simulink library "lib_IC_GFM"  (R2026a)
settings: Solver=VariableStepAuto
undefined symbols (not defined in the file): block_buses, block_buses_DC, block_idx, block_toM, buses_lf, fb, fref, iC, invL, iR, iTf, Kic, Kiv, Kpc, Kpv, Nbuses_DC, omegab, op_intconv_GFM
libraries: simulink x4, sl_discontinuities x2
(part 2 of 2)

== system lib_IC_GFM/intconv_GFM/VCC/dynamic/RC/static omega ==
  i_d_in : Inport
  i_d_out : Inport  Port=2
  i_q_in : Inport  Port=3
  i_q_out : Inport  Port=4
  Gain : Gain  Gain=1./(iR.^2+C.^2)
  Gain2 : Gain  Gain=1./(iR.^2+C.^2)
  Gain3 : Gain  Gain=iR
  Gain4 : Gain  Gain=C
  Gain5 : Gain  Gain=iR
  Gain6 : Gain  Gain=C
  Sum : Sum  Inputs=|++
  Sum1 : Sum  Inputs=|+-
  Sum2 : Sum  Inputs=|+-
  Sum4 : Sum  Inputs=|-+
  v_d : Outport
  v_q : Outport  Port=2
  wires:
  Sum/1 -> v_d/1
  Sum4/1 -> v_q/1
  Gain5/1 -> Sum4/2
  Gain4/1 -> Sum4/1
  Gain6/1 -> Sum/2
  Gain3/1 -> Sum/1
  Gain2/1 -> Gain5/1, Gain6/1
  Gain/1 -> Gain3/1, Gain4/1
  i_d_out/1 -> Sum1/2
  i_d_in/1 -> Sum1/1  "id"
  i_q_out/1 -> Sum2/2  "iq2"
  Sum2/1 -> Gain2/1  "iq"
  Sum1/1 -> Gain/1  "id"
  i_q_in/1 -> Sum2/1  "iq1"

== system lib_IC_GFM/intconv_GFM/VCC/dynamic/RL/dynamic ==
  v_in_d : Inport
  v_out_d : Inport  Port=2
  v_in_q : Inport  Port=3
  v_out_q : Inport  Port=4
  Gain1 : Gain  Gain=L
  Gain2 : Gain  Gain=R
  Gain3 : Gain  Gain=R
  Gain4 : Gain  Gain=L
  Gain5 : Gain  Gain=invL.*omegab
  Gain7 : Gain  Gain=invL.*omegab
  Product : Product
  Product1 : Product
  Sum4 : Sum  Inputs=+-|
  Sum5 : Sum  Inputs=|-+
  Sum6 : Sum  Inputs=|++
  Sum7 : Sum  Inputs=-+|
  Sum8 : Sum  Inputs=|+-
  Sum9 : Sum  Inputs=-+|
  i_d : Integrator  InitialCondition=op_intconv_GFM.VCC_dynamic_RL_dynamic_i_d
  i_q : Integrator  InitialCondition=op_intconv_GFM.VCC_dynamic_RL_dynamic_i_q
  id : Outport
  iq : Outport  Port=2
  wires:
  v_in_q/1 -> Sum5/2  "v_in_q"
  v_in_d/1 -> Sum4/1  "v_in_d"
  Gain2/1 -> Sum4/2
  i_d/1 -> Gain2/1, Gain1/1, id/1  "id"
  Sum6/1 -> Gain5/1
  [omega_ref] -> Product1/1, Product/2  "omega"
  Gain5/1 -> i_d/1
  Product/1 -> Sum6/2
  Sum8/1 -> Gain7/1
  Sum4/1 -> Sum7/2
  Product1/1 -> Sum8/2
  Gain4/1 -> Product/1
  Sum7/1 -> Sum6/1
  Gain3/1 -> Sum5/1
  Sum5/1 -> Sum9/2
  Gain7/1 -> i_q/1
  i_q/1 -> Gain3/1, Gain4/1, iq/1  "iq"
  Gain1/1 -> Product1/2
  Sum9/1 -> Sum8/1
  v_out_d/1 -> Sum7/1  "v_out_d"
  v_out_q/1 -> Sum9/1  "v_out_q"

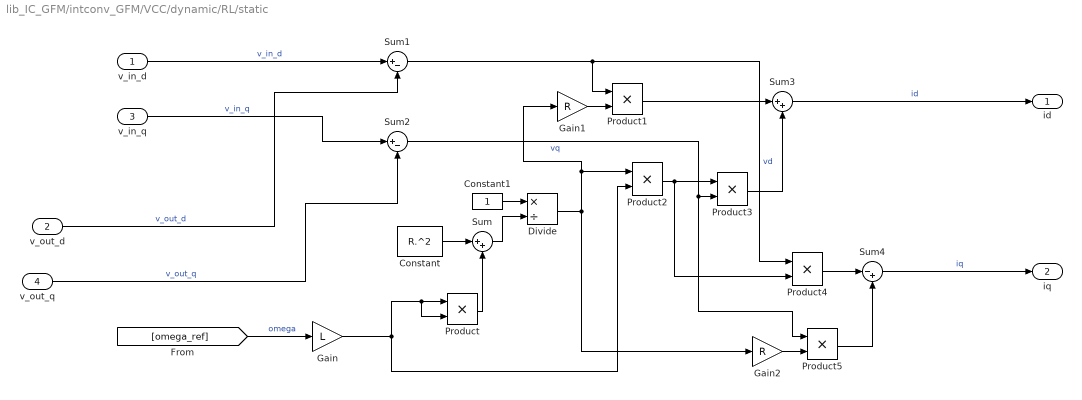
== system lib_IC_GFM/intconv_GFM/VCC/dynamic/RL/static ==
  v_in_d : Inport
  v_out_d : Inport  Port=2
  v_in_q : Inport  Port=3
  v_out_q : Inport  Port=4
  Constant : Constant  Value=R.^2
  Constant1 : Constant
  Divide : Product  Inputs=*/
  Gain : Gain  Gain=L
  Gain1 : Gain  Gain=R
  Gain2 : Gain  Gain=R
  Product{,1..5} (6 alike) : Product
  Sum : Sum  Inputs=|++
  Sum1 : Sum  Inputs=|+-
  Sum2 : Sum  Inputs=|+-
  Sum3 : Sum  Inputs=|++
  Sum4 : Sum  Inputs=|-+
  id : Outport
  iq : Outport  Port=2
  wires:
  v_in_q/1 -> Sum2/1  "v_in_q"
  v_out_d/1 -> Sum1/2  "v_out_d"
  Sum/1 -> Divide/2
  Gain2/1 -> Product5/2
  Product/1 -> Sum/2
  Product1/1 -> Sum3/1
  Product5/1 -> Sum4/2
  Constant/1 -> Sum/1
  Sum2/1 -> Product3/2, Product5/1  "vq"
  Gain/1 -> Product2/2, Product/1, Product/2
  Constant1/1 -> Divide/1
  Product3/1 -> Sum3/2
  Sum1/1 -> Product4/1, Product1/1  "vd"
  Divide/1 -> Product2/1, Gain1/1, Gain2/1
  Product4/1 -> Sum4/1
  Product2/1 -> Product3/1, Product4/2
  Gain1/1 -> Product1/2
  Sum3/1 -> id/1  "id"
  Sum4/1 -> iq/1  "iq"
  v_out_q/1 -> Sum2/2  "v_out_q"
  v_in_d/1 -> Sum1/1  "v_in_d"
  [omega_ref] -> Gain/1  "omega"

== system lib_IC_GFM/intconv_GFM/VCC/dynamic/RL/static_omega ==
  v_in_d : Inport
  v_out_d : Inport  Port=2
  v_in_q : Inport  Port=3
  v_out_q : Inport  Port=4
  Gain : Gain  Gain=1./(R.^2+L.^2)
  Gain2 : Gain  Gain=1./(R.^2+L.^2)
  Gain3 : Gain  Gain=R
  Gain4 : Gain  Gain=L
  Gain5 : Gain  Gain=L
  Gain6 : Gain  Gain=R
  Sum : Sum  Inputs=|++
  Sum1 : Sum  Inputs=|+-
  Sum2 : Sum  Inputs=|+-
  Sum3 : Sum  Inputs=|-+
  id : Outport
  iq : Outport  Port=2
  wires:
  Gain6/1 -> Sum3/2
  Sum3/1 -> iq/1
  Gain5/1 -> Sum3/1
  Sum/1 -> id/1
  Gain2/1 -> Gain4/1, Gain6/1
  Gain4/1 -> Sum/2
  Gain3/1 -> Sum/1
  Gain/1 -> Gain3/1, Gain5/1
  Sum2/1 -> Gain2/1  "vq"
  Sum1/1 -> Gain/1  "vd"
  v_out_d/1 -> Sum1/2  "v_out_d"
  v_out_q/1 -> Sum2/2  "v_out_q"
  v_in_d/1 -> Sum1/1  "v_in_d"
  v_in_q/1 -> Sum2/1  "v_in_q"

== system lib_IC_GFM/intconv_GFM/VCC/dynamic_VC/RC/dynamic ==
  omega : Inport
  i_d_in : Inport  Port=2
  i_d_out : Inport  Port=3
  i_q_in : Inport  Port=4
  i_q_out : Inport  Port=5
  Gain1 : Gain  Gain=iR
  Gain2 : Gain  Gain=iR
  Gain3 : Gain  Gain=C
  Gain4 : Gain  Gain=C
  Gain5 : Gain  Gain=iC.*omegab
  Gain6 : Gain  Gain=iC.*omegab
  Product : Product
  Product1 : Product
  Sum10 : Sum  Inputs=|-++
  Sum11 : Sum  Inputs=-+|
  Sum12 : Sum  Inputs=|+-
  Sum13 : Sum  Inputs=-+-|
  vd : Integrator  InitialCondition=op_intconv_GFM.VCC_dynamic_VC_RC_dynamic_vd
  vq : Integrator  InitialCondition=op_intconv_GFM.VCC_dynamic_VC_RC_dynamic_vq
  v_d : Outport
  v_q : Outport  Port=2
  wires:
  i_q_out/1 -> Sum12/2  "iq2"
  i_q_in/1 -> Sum12/1  "iq1"
  i_d_out/1 -> Sum11/1  "id2"
  i_d_in/1 -> Sum11/2  "id1"
  vd/1 -> Gain1/1, v_d/1, Gain4/1  "vd"
  Sum12/1 -> Sum13/2
  Gain5/1 -> vq/1
  Gain1/1 -> Sum10/1
  Sum13/1 -> Gain5/1
  omega/1 -> Product1/2, Product/2  "omega"
  Gain6/1 -> vd/1
  Sum11/1 -> Sum10/2
  Product/1 -> Sum13/1
  Gain2/1 -> Sum13/3
  Gain4/1 -> Product/1
  Product1/1 -> Sum10/3
  vq/1 -> Gain3/1, Gain2/1, v_q/1  "vq"
  Gain3/1 -> Product1/1
  Sum10/1 -> Gain6/1

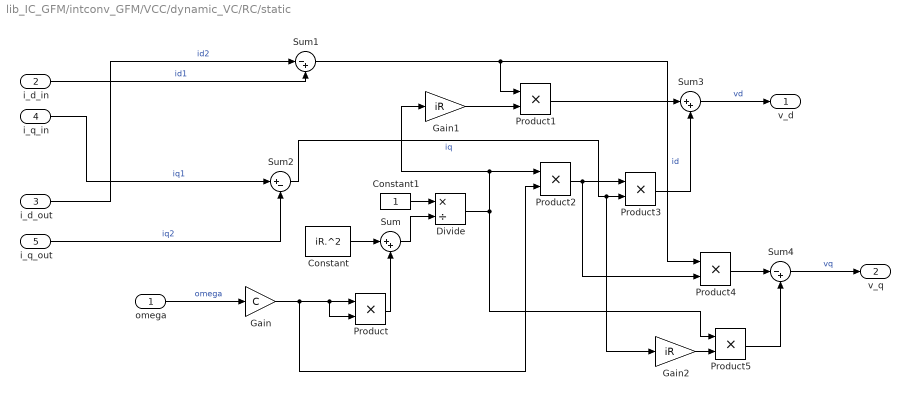
== system lib_IC_GFM/intconv_GFM/VCC/dynamic_VC/RC/static ==
  omega : Inport
  i_d_in : Inport  Port=2
  i_d_out : Inport  Port=3
  i_q_in : Inport  Port=4
  i_q_out : Inport  Port=5
  Constant : Constant  Value=iR.^2
  Constant1 : Constant
  Divide : Product  Inputs=*/
  Gain : Gain  Gain=C
  Gain1 : Gain  Gain=iR
  Gain2 : Gain  Gain=iR
  Product{,1..5} (6 alike) : Product
  Sum : Sum  Inputs=|++
  Sum1 : Sum  Inputs=|-+
  Sum2 : Sum  Inputs=|+-
  Sum3 : Sum  Inputs=|++
  Sum4 : Sum  Inputs=|-+
  v_d : Outport
  v_q : Outport  Port=2
  wires:
  i_q_out/1 -> Sum2/2  "iq2"
  i_q_in/1 -> Sum2/1  "iq1"
  i_d_out/1 -> Sum1/1  "id2"
  i_d_in/1 -> Sum1/2  "id1"
  omega/1 -> Gain/1  "omega"
  Sum3/1 -> v_d/1  "vd"
  Sum4/1 -> v_q/1  "vq"
  Constant/1 -> Sum/1
  Sum/1 -> Divide/2
  Gain/1 -> Product2/2, Product/2, Product/1
  Product/1 -> Sum/2
  Constant1/1 -> Divide/1
  Sum1/1 -> Product1/1, Product4/1  "id"
  Sum2/1 -> Gain2/1, Product3/2  "iq"
  Gain1/1 -> Product1/2
  Divide/1 -> Product5/1, Gain1/1, Product2/1
  Product1/1 -> Sum3/1
  Product3/1 -> Sum3/2
  Product2/1 -> Product4/2, Product3/1
  Product4/1 -> Sum4/1
  Gain2/1 -> Product5/2
  Product5/1 -> Sum4/2

== system lib_IC_GFM/intconv_GFM/VCC/dynamic_VC/RC/static omega ==
  i_d_in : Inport
  i_d_out : Inport  Port=2
  i_q_in : Inport  Port=3
  i_q_out : Inport  Port=4
  Gain : Gain  Gain=1./(iR.^2+C.^2)
  Gain2 : Gain  Gain=1./(iR.^2+C.^2)
  Gain3 : Gain  Gain=iR
  Gain4 : Gain  Gain=C
  Gain5 : Gain  Gain=iR
  Gain6 : Gain  Gain=C
  Sum : Sum  Inputs=|++
  Sum1 : Sum  Inputs=|+-
  Sum2 : Sum  Inputs=|+-
  Sum4 : Sum  Inputs=|-+
  v_d : Outport
  v_q : Outport  Port=2
  wires:
  Sum/1 -> v_d/1
  Sum4/1 -> v_q/1
  Gain5/1 -> Sum4/2
  Gain4/1 -> Sum4/1
  Gain6/1 -> Sum/2
  Gain3/1 -> Sum/1
  Gain2/1 -> Gain5/1, Gain6/1
  Gain/1 -> Gain3/1, Gain4/1
  i_d_out/1 -> Sum1/2
  i_d_in/1 -> Sum1/1  "id"
  i_q_out/1 -> Sum2/2  "iq2"
  Sum2/1 -> Gain2/1  "iq"
  Sum1/1 -> Gain/1  "id"
  i_q_in/1 -> Sum2/1  "iq1"

== system lib_IC_GFM/intconv_GFM/VCC/dynamic_limiting/RC/dynamic ==
  omega : Inport
  i_d_in : Inport  Port=2
  i_d_out : Inport  Port=3
  i_q_in : Inport  Port=4
  i_q_out : Inport  Port=5
  Gain1 : Gain  Gain=iR
  Gain2 : Gain  Gain=iR
  Gain3 : Gain  Gain=C
  Gain4 : Gain  Gain=C
  Gain5 : Gain  Gain=iC.*omegab
  Gain6 : Gain  Gain=iC.*omegab
  Product : Product
  Product1 : Product
  Sum10 : Sum  Inputs=|-++
  Sum11 : Sum  Inputs=-+|
  Sum12 : Sum  Inputs=|+-
  Sum13 : Sum  Inputs=-+-|
  vd : Integrator  InitialCondition=op_intconv_GFM.VCC_dynamic_limiting_RC_dynamic_vd
  vq : Integrator  InitialCondition=op_intconv_GFM.VCC_dynamic_limiting_RC_dynamic_vq
  v_d : Outport
  v_q : Outport  Port=2
  wires:
  Sum10/1 -> Gain6/1
  Gain3/1 -> Product1/1
  vq/1 -> v_q/1, Gain2/1, Gain3/1  "vq"
  Product1/1 -> Sum10/3
  Gain4/1 -> Product/1
  Gain2/1 -> Sum13/3
  Product/1 -> Sum13/1
  Sum11/1 -> Sum10/2
  Gain6/1 -> vd/1
  omega/1 -> Product/2, Product1/2  "omega"
  Sum13/1 -> Gain5/1
  Gain1/1 -> Sum10/1
  Gain5/1 -> vq/1
  Sum12/1 -> Sum13/2
  vd/1 -> Gain4/1, v_d/1, Gain1/1  "vd"
  i_d_in/1 -> Sum11/2  "id1"
  i_d_out/1 -> Sum11/1  "id2"
  i_q_in/1 -> Sum12/1  "iq1"
  i_q_out/1 -> Sum12/2  "iq2"

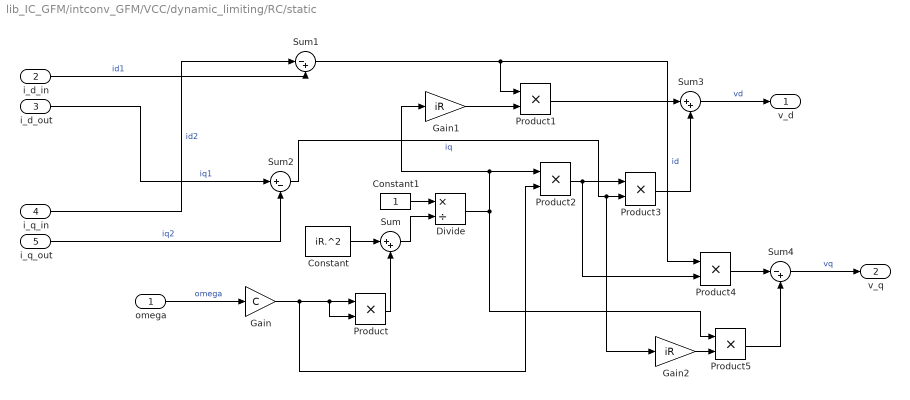
== system lib_IC_GFM/intconv_GFM/VCC/dynamic_limiting/RC/static ==
  omega : Inport
  i_d_in : Inport  Port=2
  i_d_out : Inport  Port=3
  i_q_in : Inport  Port=4
  i_q_out : Inport  Port=5
  Constant : Constant  Value=iR.^2
  Constant1 : Constant
  Divide : Product  Inputs=*/
  Gain : Gain  Gain=C
  Gain1 : Gain  Gain=iR
  Gain2 : Gain  Gain=iR
  Product{,1..5} (6 alike) : Product
  Sum : Sum  Inputs=|++
  Sum1 : Sum  Inputs=|-+
  Sum2 : Sum  Inputs=|+-
  Sum3 : Sum  Inputs=|++
  Sum4 : Sum  Inputs=|-+
  v_d : Outport
  v_q : Outport  Port=2
  wires:
  Product5/1 -> Sum4/2
  Gain2/1 -> Product5/2
  Product4/1 -> Sum4/1
  Product2/1 -> Product3/1, Product4/2
  Product3/1 -> Sum3/2
  Product1/1 -> Sum3/1
  Divide/1 -> Product2/1, Gain1/1, Product5/1
  Gain1/1 -> Product1/2
  Sum2/1 -> Product3/2, Gain2/1  "iq"
  Sum1/1 -> Product4/1, Product1/1  "id"
  Constant1/1 -> Divide/1
  Product/1 -> Sum/2
  Gain/1 -> Product/1, Product/2, Product2/2
  Sum/1 -> Divide/2
  Constant/1 -> Sum/1
  Sum4/1 -> v_q/1  "vq"
  Sum3/1 -> v_d/1  "vd"
  omega/1 -> Gain/1  "omega"
  i_d_in/1 -> Sum1/2  "id1"
  i_q_in/1 -> Sum1/1  "id2"
  i_d_out/1 -> Sum2/1  "iq1"
  i_q_out/1 -> Sum2/2  "iq2"

== system lib_IC_GFM/intconv_GFM/VCC/dynamic_limiting/RC/static omega ==
  i_d_in : Inport
  i_d_out : Inport  Port=2
  i_q_in : Inport  Port=3
  i_q_out : Inport  Port=4
  Gain : Gain  Gain=1./(iR.^2+C.^2)
  Gain2 : Gain  Gain=1./(iR.^2+C.^2)
  Gain3 : Gain  Gain=iR
  Gain4 : Gain  Gain=C
  Gain5 : Gain  Gain=iR
  Gain6 : Gain  Gain=C
  Sum : Sum  Inputs=|++
  Sum1 : Sum  Inputs=|+-
  Sum2 : Sum  Inputs=|+-
  Sum4 : Sum  Inputs=|-+
  v_d : Outport
  v_q : Outport  Port=2
  wires:
  i_q_in/1 -> Sum2/1  "iq1"
  Sum1/1 -> Gain/1  "id"
  Sum2/1 -> Gain2/1  "iq"
  i_q_out/1 -> Sum2/2  "iq2"
  i_d_in/1 -> Sum1/1  "id"
  i_d_out/1 -> Sum1/2
  Gain/1 -> Gain4/1, Gain3/1
  Gain2/1 -> Gain6/1, Gain5/1
  Gain3/1 -> Sum/1
  Gain6/1 -> Sum/2
  Gain4/1 -> Sum4/1
  Gain5/1 -> Sum4/2
  Sum4/1 -> v_q/1
  Sum/1 -> v_d/1

== system lib_IC_GFM/intconv_GFM/VCC/dynamic_limiting/RL/dynamic ==
  v_in_d : Inport
  v_out_d : Inport  Port=2
  v_in_q : Inport  Port=3
  v_out_q : Inport  Port=4
  Gain1 : Gain  Gain=L
  Gain2 : Gain  Gain=R
  Gain3 : Gain  Gain=R
  Gain4 : Gain  Gain=L
  Gain5 : Gain  Gain=invL.*omegab
  Gain7 : Gain  Gain=invL.*omegab
  Product : Product
  Product1 : Product
  Sum4 : Sum  Inputs=+-|
  Sum5 : Sum  Inputs=|-+
  Sum6 : Sum  Inputs=|++
  Sum7 : Sum  Inputs=-+|
  Sum8 : Sum  Inputs=|+-
  Sum9 : Sum  Inputs=-+|
  i_d : Integrator  InitialCondition=op_intconv_GFM.VCC_dynamic_limiting_RL_dynamic_i_d
  i_q : Integrator  InitialCondition=op_intconv_GFM.VCC_dynamic_limiting_RL_dynamic_i_q
  id : Outport
  iq : Outport  Port=2
  wires:
  v_out_q/1 -> Sum9/1  "v_out_q"
  v_out_d/1 -> Sum7/1  "v_out_d"
  Sum9/1 -> Sum8/1
  Gain1/1 -> Product1/2
  i_q/1 -> iq/1, Gain4/1, Gain3/1  "iq"
  Gain7/1 -> i_q/1
  Sum5/1 -> Sum9/2
  Gain3/1 -> Sum5/1
  Sum7/1 -> Sum6/1
  Gain4/1 -> Product/1
  Product1/1 -> Sum8/2
  Sum4/1 -> Sum7/2
  Sum8/1 -> Gain7/1
  Product/1 -> Sum6/2
  Gain5/1 -> i_d/1
  [omega_leader_VCVSC] -> Product/2, Product1/1  "omega"
  Sum6/1 -> Gain5/1
  i_d/1 -> id/1, Gain1/1, Gain2/1  "id"
  Gain2/1 -> Sum4/2
  v_in_d/1 -> Sum4/1  "v_in_d"
  v_in_q/1 -> Sum5/2  "v_in_q"

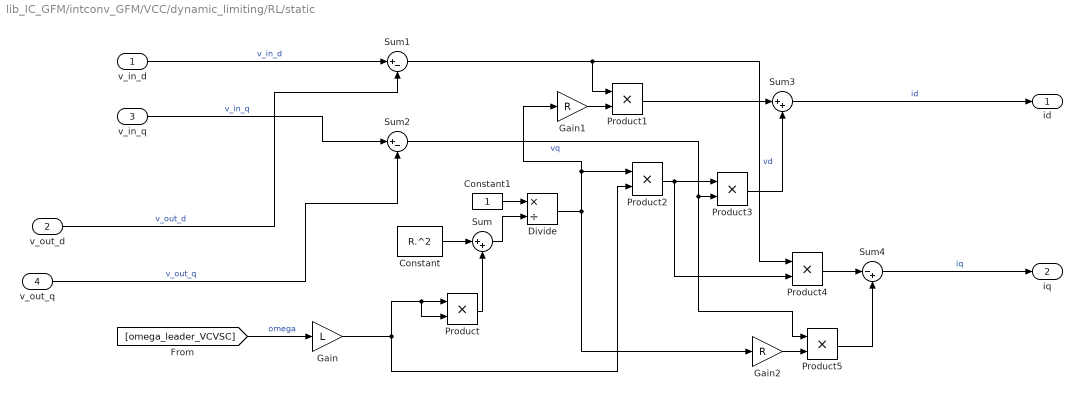
== system lib_IC_GFM/intconv_GFM/VCC/dynamic_limiting/RL/static ==
  v_in_d : Inport
  v_out_d : Inport  Port=2
  v_in_q : Inport  Port=3
  v_out_q : Inport  Port=4
  Constant : Constant  Value=R.^2
  Constant1 : Constant
  Divide : Product  Inputs=*/
  Gain : Gain  Gain=L
  Gain1 : Gain  Gain=R
  Gain2 : Gain  Gain=R
  Product{,1..5} (6 alike) : Product
  Sum : Sum  Inputs=|++
  Sum1 : Sum  Inputs=|+-
  Sum2 : Sum  Inputs=|+-
  Sum3 : Sum  Inputs=|++
  Sum4 : Sum  Inputs=|-+
  id : Outport
  iq : Outport  Port=2
  wires:
  [omega_leader_VCVSC] -> Gain/1  "omega"
  v_in_d/1 -> Sum1/1  "v_in_d"
  v_out_q/1 -> Sum2/2  "v_out_q"
  Sum4/1 -> iq/1  "iq"
  Sum3/1 -> id/1  "id"
  Gain1/1 -> Product1/2
  Product2/1 -> Product4/2, Product3/1
  Product4/1 -> Sum4/1
  Divide/1 -> Gain2/1, Gain1/1, Product2/1
  Sum1/1 -> Product1/1, Product4/1  "vd"
  Product3/1 -> Sum3/2
  Constant1/1 -> Divide/1
  Gain/1 -> Product/2, Product/1, Product2/2
  Sum2/1 -> Product5/1, Product3/2  "vq"
  Constant/1 -> Sum/1
  Product5/1 -> Sum4/2
  Product1/1 -> Sum3/1
  Product/1 -> Sum/2
  Gain2/1 -> Product5/2
  Sum/1 -> Divide/2
  v_out_d/1 -> Sum1/2  "v_out_d"
  v_in_q/1 -> Sum2/1  "v_in_q"

== system lib_IC_GFM/intconv_GFM/VCC/dynamic_limiting/RL/static_omega ==
  v_in_d : Inport
  v_out_d : Inport  Port=2
  v_in_q : Inport  Port=3
  v_out_q : Inport  Port=4
  Gain : Gain  Gain=1./(R.^2+L.^2)
  Gain2 : Gain  Gain=1./(R.^2+L.^2)
  Gain3 : Gain  Gain=R
  Gain4 : Gain  Gain=L
  Gain5 : Gain  Gain=L
  Gain6 : Gain  Gain=R
  Sum : Sum  Inputs=|++
  Sum1 : Sum  Inputs=|+-
  Sum2 : Sum  Inputs=|+-
  Sum3 : Sum  Inputs=|-+
  id : Outport
  iq : Outport  Port=2
  wires:
  v_in_q/1 -> Sum2/1  "v_in_q"
  v_in_d/1 -> Sum1/1  "v_in_d"
  v_out_q/1 -> Sum2/2  "v_out_q"
  v_out_d/1 -> Sum1/2  "v_out_d"
  Sum1/1 -> Gain/1  "vd"
  Sum2/1 -> Gain2/1  "vq"
  Gain/1 -> Gain5/1, Gain3/1
  Gain3/1 -> Sum/1
  Gain4/1 -> Sum/2
  Gain2/1 -> Gain6/1, Gain4/1
  Sum/1 -> id/1
  Gain5/1 -> Sum3/1
  Sum3/1 -> iq/1
  Gain6/1 -> Sum3/2

== system lib_IC_GFM/intconv_GFM/VI/WOF_d/Active/Impl ==
  In1 : Inport
  Gain : Gain  Gain=iTf
  I : Integrator  InitialConditionSource=external  InitialCondition=op_intconv_GFM.VI_WOF_d_Active_Impl_I
  Sum : Sum  Inputs=+-|
  Sum4 : Sum  Inputs=|+-
  Out1 : Outport
  wires:
  Sum/1 -> Out1/1
  I/1 -> Sum4/2, Sum/2
  In1/1 -> Sum4/1, Sum/1, I/2
  Sum4/1 -> Gain/1
  Gain/1 -> I/1

== system lib_IC_GFM/intconv_GFM/VI/WOF_q/Active/Impl ==
  In1 : Inport
  Gain : Gain  Gain=iTf
  I : Integrator  InitialConditionSource=external  InitialCondition=op_intconv_GFM.VI_WOF_q_Active_Impl_I
  Sum : Sum  Inputs=+-|
  Sum4 : Sum  Inputs=|+-
  Out1 : Outport
  wires:
  Sum/1 -> Out1/1
  I/1 -> Sum4/2, Sum/2
  In1/1 -> Sum4/1, Sum/1, I/2
  Sum4/1 -> Gain/1
  Gain/1 -> I/1

== matlab function lib_IC_GFM/intconv_GFM/Gen_To_DC ==
  data: u input; y output; Nbuses_DC parameter; block_buses_DC parameter
function y = fcn(u, Nbuses_DC, block_buses_DC)

y = zeros(1, Nbuses_DC);
for i=1:Nbuses_DC
    y(i) = sum(u(block_buses_DC == i));
end
